simulink model "DiscreteTimeIntegrator"  (R2026b)
settings: Solver=VariableStepAuto
values from neighbouring files (symbols this model uses):
  Ts = 1e-5    (= 1e-05)    [coeficientes.m]
settings Model: Creator=fedeb  LastModifiedBy=fedeb

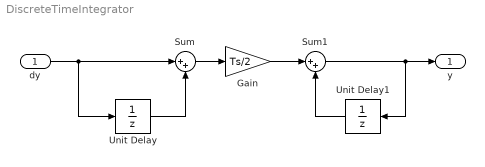
== system DiscreteTimeIntegrator ==
  dy : Inport
  Gain : Gain  Gain=Ts/2
  Sum : Sum  Inputs=|++
  Sum1 : Sum  Inputs=|++
  Unit Delay : UnitDelay  SampleTime=Ts
  Unit Delay1 : UnitDelay  SampleTime=Ts
  y : Outport
  wires:
  dy/1 -> Sum/1, Unit Delay/1
  Unit Delay/1 -> Sum/2
  Sum/1 -> Gain/1
  Gain/1 -> Sum1/1
  Sum1/1 -> Unit Delay1/1, y/1
  Unit Delay1/1 -> Sum1/2
